simulink model "position_velocity_cascade"  (R2025b)
settings: configuration reference "MCConfiguration" (kept outside this file)
model workspace (MAT data in the model file):
  ControlOuter_Ts = Simulink.Parameter
  ControlOuter_Ts.Value = 0.001
  ControlOuter_Ts.Complexity = 'real'
  ControlOuter_Ts.Dimensions = [1 1]
  ControlOuter_Ts.DataType = 'auto'
  ControlOuter_Ts.DocUnits = 's'
undefined symbols (not defined in the file): ControlModes, DiscIntNeverNeededParam
libraries: simulink x12, slpidlib x3, simulink_extras x1
settings Model: DataDictionary=embeddedBoard_common.sldd  Creator=ascalzo  LastModifiedBy=rpumpo
settings ConfigSetRef: SourceName=MCConfiguration

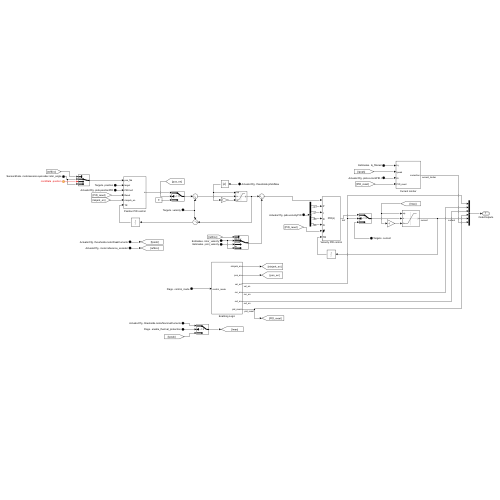
[thumbnail: Simulink's stored preview of the top-level diagram]
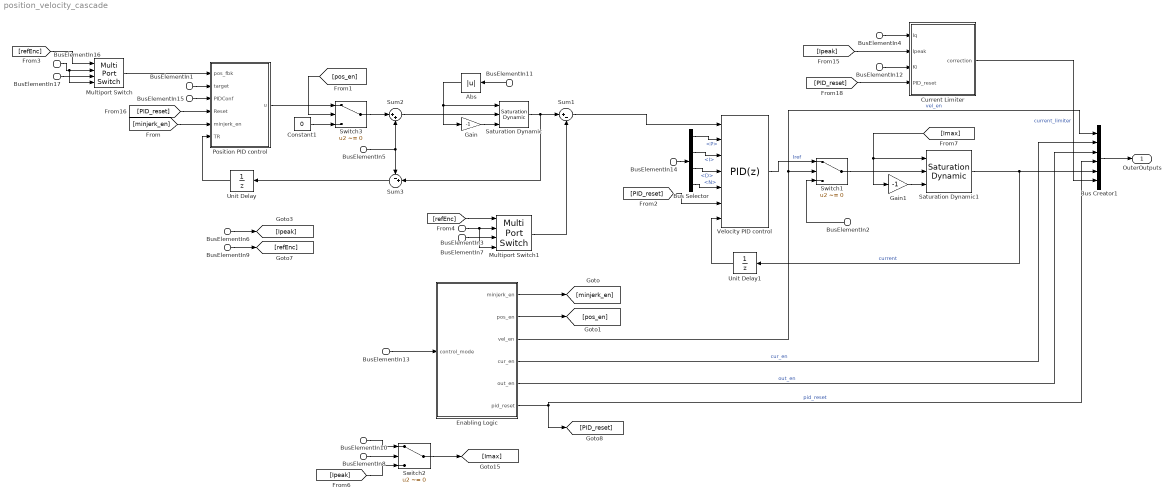
== system position_velocity_cascade ==
  BusElementIn3 : Inport  Description=velocity  PortName=Estimates  Element=rotor_velocity
  BusElementIn4 : Inport  Description=filtered motor current  PortName=Estimates  Element=Iq_filtered
  BusElementIn7 : Inport  Description=velocity  PortName=Estimates  Element=joint_velocity
  BusElementIn1 : Inport  Port=2  PortName=Targets  Element=position
  BusElementIn5 : Inport  Port=2  PortName=Targets  Element=velocity
  BusElementIn2 : Inport  Port=2  PortName=Targets  Element=current
  BusElementIn17 : Inport  Description=position encoder after gearbox  Port=3  PortName=JointData  Element=position
  BusElementIn11 : Inport  Description=Can be only non-negative  Port=4  PortName=ActuatorCfg  Element=thresholds.jntVelMax
  BusElementIn10 : Inport  Description=|  Port=4  PortName=ActuatorCfg  Element=thresholds.motorNominalCurrents
      | Current that can be kept for an indefinite period of time w/o damaging the motor
      | Expressed in [A] as all the internal computations are done this way
      | Can be only non-negative
  BusElementIn6 : Inport  Description=|  Port=4  PortName=ActuatorCfg  Element=thresholds.motorPeakCurrents
      | Current that can be applied for a short period of time
      | Expressed in [A] as all the internal computations are done this way
      | Can be only non-negative
  BusElementIn12 : Inport  Port=4  PortName=ActuatorCfg  Element=pids.currentPID.I
  BusElementIn14 : Inport  Port=4  PortName=ActuatorCfg  Element=pids.velocityPID
  BusElementIn15 : Inport  Port=4  PortName=ActuatorCfg  Element=pids.positionPID
  BusElementIn9 : Inport  Port=4  PortName=ActuatorCfg  Element=motor.reference_encoder
  BusElementIn16 : Inport  Description=Mechanical Angle before gearbox  Port=5  PortName=SensorsData  Element=motorsensors.qencoder.rotor_angle
  BusElementIn8 : Inport  Port=6  PortName=Flags  Element=enable_thermal_protection
  BusElementIn13 : Inport  Description=control mode  Port=6  PortName=Flags  Element=control_mode
  Abs : Abs  SaturateOnIntegerOverflow=off
  Bus Creator1 : BusCreator  Inputs=6  OutDataTypeStr=Bus: ControlOuterOutputs  NonVirtualBus=on
      settings: InheritFromInputs=off
  Bus Selector : BusSelector  OutputSignals=P,I,D,N
  Constant1 : Constant  Value=0  OutDataTypeStr=single  SampleTime=-1
  Current Limiter : Subsystem
  Enabling Logic : Subsystem
      settings: PortSchema="{\"entries\":[{\"content\":{\"sides\":[{\"content\":{},\"type\":\"ConnectorPlacement.EquallySpacedRectSide\",\"uuid\":\"90c86a81-f753-4d73-9375-c811c35622e9\"},{\"content\":{\"side\":\"RIGHT\"},\"type\":\"ConnectorPlacement.EquallySpacedRectSide\",\"uuid\":\"e17254f2-3c2d-4692-9f9e-d71cfac23eea\"},{\"content\":{\"connectorIds\":[\"Out1\",\"Out2\",\"Out3\",\"Out4\",\"Out5\",\"Out6\"],\"side\":\"TOP\"},\"type\":\"ConnectorPlacement.EquallySpacedRectSide\",\"uuid\":\"448c88e2-24ce-4de3-becf-cb98b7ef78f6\"},{\"content\":{\"connectorIds\":[\"In1\"],\"side\":\"BOTTOM\"},\"type\":\"ConnectorPlacement.EquallySpacedRectSide\",\"uuid\":\"8605ddaa-364c-411c-83c1-7277cb4d54d2\"}]},\"type\":\"ConnectorPlacement.EquallySpacedConnector\",\"uuid\":\"c1415ecc-9e2a-4576-ac3b-1f6784fd4a23\"}],\"packageUris\":[\"http://schema.mathworks.com/mf0/Connector/R2020b\"],\"version\":\"1.0\"}"
  Gain : Gain  Gain=-1
  Gain1 : Gain  Gain=-1
  Multiport Switch : MultiPortSwitch  DataPortOrder=Specify indices  Inputs=2  DataPortIndices={ ReferenceEncoder.Motor, ReferenceEncoder.Joint}  DataPortForDefault=Additional data port  SaturateOnIntegerOverflow=off  InputSameDT=off
  Multiport Switch1 : MultiPortSwitch  DataPortOrder=Specify indices  Inputs=2  DataPortIndices={ ReferenceEncoder.Motor, ReferenceEncoder.Joint}  DataPortForDefault=Additional data port  SaturateOnIntegerOverflow=off  InputSameDT=off
  Position PID control : Subsystem
  Saturation Dynamic : simulink/Discontinuities/Saturation Dynamic  OutMin=[]  OutMax=[]  OutDataTypeStr=Inherit: Same as second input  OutDataType=fixdt(1, 16)  OutScaling=2^-10  DoSatur=off
  Saturation Dynamic1 : simulink/Discontinuities/Saturation Dynamic  OutMin=[]  OutMax=[]  OutDataTypeStr=Inherit: Same as second input  OutDataType=fixdt(1, 16)  OutScaling=2^-10  DoSatur=off
  Sum1 : Sum  Inputs=|+-
  Sum2 : Sum  Inputs=|++
  Sum3 : Sum  Inputs=-+|
  Switch1 : Switch  Criteria=u2 ~= 0  SaturateOnIntegerOverflow=off  InputSameDT=off
  Switch2 : Switch  Criteria=u2 ~= 0  SaturateOnIntegerOverflow=off  InputSameDT=off
  Switch3 : Switch  Criteria=u2 ~= 0  SaturateOnIntegerOverflow=off  InputSameDT=off
  Unit Delay : UnitDelay  SampleTime=-1  HasFrameUpgradeWarning=on
  Unit Delay1 : UnitDelay  SampleTime=-1  HasFrameUpgradeWarning=on
  Velocity PID control : slpidlib/PID Controller  Controller=PID  Form=Parallel  TimeDomain=Discrete-time  UseExternalTs=off  SampleTime=-1  IntegratorMethod=Trapezoidal  FilterMethod=Trapezoidal  ControllerParametersSource=external  P=100  I=0  UseKiTs=off  D=0  UseExternalDerivativeSource=off  N=100  UseFilter=on  TunerSelectOption=Frequency Response Based  InitialConditionSource=internal  InitialConditionForIntegrator=0  InitialConditionForFilter=0  DifferentiatorICPrevScaledInput=0  ExternalReset=rising  TrackingMode=on  Kt=1  LimitOutput=off  SatLimitsSource=internal  UpperSaturationLimit=100  LowerSaturationLimit=-100  LinearizeAsGain=on  AntiWindupMode=clamping  Kb=1  LimitIntegrator=off  UpperIntegratorSaturationLimit=inf  LowerIntegratorSaturationLimit=-inf  POutMin=[]  POutMax=[]  IOutMin=[]  IOutMax=[]  DOutMin=[]  DOutMax=[]  NOutMin=[]  NOutMax=[]  SumOutMin=[]  SumOutMax=[]  SaturationOutMin=[]  SaturationOutMax=[]  PParamMin=[]  PParamMax=[]  IParamMin=[]  IParamMax=[]  DParamMin=[]  DParamMax=[]  NParamMin=[]  NParamMax=[]  KbParamMin=[]  KbParamMax=[]  KtParamMin=[]  KtParamMax=[]  KbOutMin=[]  KbOutMax=[]  KtOutMin=[]  KtOutMax=[]  IntegratorOutMin=[]  IntegratorOutMax=[]  FilterOutMin=[]  FilterOutMax=[]  SumI1OutMin=[]  SumI1OutMax=[]  SumI2OutMin=[]  SumI2OutMax=[]  SumI3OutMin=[]  SumI3OutMax=[]  SumI4OutMin=[]  SumI4OutMax=[]  SumDOutMin=[]  SumDOutMax=[]  DifferentiatorOutMin=[]  DifferentiatorOutMax=[]  FilterDiffOutCoefMin=[]  FilterDiffOutCoefMax=[]  ReciprocalOutMin=[]  ReciprocalOutMax=[]  SumDenOutMin=[]  SumDenOutMax=[]  SumNumOutMin=[]  SumNumOutMax=[]  DivideOutMin=[]  DivideOutMax=[]  UdiffTsProdOutMin=[]  UdiffTsProdOutMax=[]  NTsProdOutMin=[]  NTsProdOutMax=[]  UintegralTsProdOutMin=[]  UintegralTsProdOutMax=[]  UngainTsProdOutMin=[]  UngainTsProdOutMax=[]  ClampingZeroOutDataTypeStr=Inherit: Inherit via back propagation  ClampingZeroOutMin=[]  ClampingZeroOutMax=[]  FilterDenConstantOutDataTypeStr=Inherit: Inherit via back propagation  FilterDenConstantOutMin=[]  FilterDenConstantOutMax=[]  PCopyOutDataTypeStr=Inherit: Inherit via back propagation  PCopyOutMin=[]  PCopyOutMax=[]  NCopyOutDataTypeStr=Inherit: Inherit via back propagation  NCopyOutMin=[]  NCopyOutMax=[]  IntegratorContinuousStateAttributes=''  IntegratorStateMustResolveToSignalObject=off  IntegratorRTWStateStorageClass=Auto  FilterContinuousStateAttributes=''  FilterStateMustResolveToSignalObject=off  FilterRTWStateStorageClass=Auto  ParallelPVariant=ExternalParameters  IdealPVariant=Disabled  IVariant=ExternalParameters  DVariant=ExternalParameters  IntegratorVariant=Discrete  SatVariant=Disabled  AWVariant=Passthrough  PCopyVariant=Disabled  TRVariant=Enabled  FdbkBlocksVariant=Feedback  IdealPFdbkVariant=Passthrough  SatFdbkVariant=Passthrough  DerivativeFilterVariant=TrapezoidalFilter  NVariant=ExternalParameters  NCopyVariant=ExternalParameters  FilterICVariant=InternalICsFilter  IntegratorICVariant=InternalICs  ExternalResetVariant=ExternalReset  TRSumVariant=TrackingMode  SumFdbkVariant=Enabled  SumVariant=Sum_PID  TsampFilterVariant=InternalTs  TsampNgainVariant=Passthrough  TsampIntegralVariant=Disabled_SignalSpec  ExternalSaturationOutDataTypeStr=Inherit: Same as second input  DerivativeSourceVariant=ErrorSignal  PreIntVariant=InternalPreInt
  OuterOutputs : Outport  OutDataTypeStr=Bus: ControlOuterOutputs  BusOutputAsStruct=on
  wires:
  [PID_reset] -> Velocity PID control/6
  BusElementIn14/1 -> Bus Selector/1
  Sum2/1 -> Saturation Dynamic/2
  Switch3/1 -> Sum2/1
  Constant1/1 -> Switch3/3
  BusElementIn15/1 -> Position PID control/3(PIDConf)
  BusElementIn1/1 -> Position PID control/2(target)
  [PID_reset] -> Position PID control/4(Reset)
  Position PID control/1(u) -> Switch3/1
  BusElementIn5/1 -> Sum3/1, Sum2/2
  Saturation Dynamic/1 -> Sum1/1, Sum3/2
  Sum3/1 -> Unit Delay/1
  Unit Delay/1 -> Position PID control/6(TR)
  Enabling Logic/1(minjerk_en) -> [minjerk_en]
  Enabling Logic/2(pos_en) -> [pos_en]
  [minjerk_en] -> Position PID control/5(minjerk_en)
  [pos_en] -> Switch3/2
  Enabling Logic/3(vel_en) -> Switch1/2, Bus Creator1/1  "vel_en"
  Enabling Logic/4(cur_en) -> Bus Creator1/2  "cur_en"
  Enabling Logic/5(out_en) -> Bus Creator1/3  "out_en"
  Bus Creator1/1 -> OuterOutputs/1
  BusElementIn13/1 -> Enabling Logic/1(control_mode)
  BusElementIn11/1 -> Abs/1
  Abs/1 -> Gain/1, Saturation Dynamic/1
  Gain/1 -> Saturation Dynamic/3
  Unit Delay1/1 -> Velocity PID control/7
  Velocity PID control/1 -> Switch1/1  "Iref"
  Switch1/1 -> Saturation Dynamic1/2
  BusElementIn2/1 -> Switch1/3
  Gain1/1 -> Saturation Dynamic1/3
  [Imax] -> Saturation Dynamic1/1, Gain1/1
  BusElementIn4/1 -> Current Limiter/1(Iq)
  [Ipeak] -> Current Limiter/2(Ipeak)
  [PID_reset] -> Current Limiter/4(PID_reset)
  BusElementIn12/1 -> Current Limiter/3(Ki)
  Sum1/1 -> Velocity PID control/1
  Enabling Logic/6(pid_reset) -> Bus Creator1/4, [PID_reset]  "pid_reset"
  Saturation Dynamic1/1 -> Bus Creator1/5, Unit Delay1/1  "current"
  Current Limiter/1(correction) -> Bus Creator1/6  "current_limiter"
  [Ipeak] -> Switch2/3
  BusElementIn10/1 -> Switch2/1
  BusElementIn8/1 -> Switch2/2
  Switch2/1 -> [Imax]
  Multiport Switch/1 -> Position PID control/1(pos_fbk)
  [refEnc] -> Multiport Switch/1
  BusElementIn17/1 -> Multiport Switch/3
  BusElementIn16/1 -> Multiport Switch/4, Multiport Switch/2
  BusElementIn3/1 -> Multiport Switch1/4, Multiport Switch1/2
  BusElementIn7/1 -> Multiport Switch1/3
  Multiport Switch1/1 -> Sum1/2
  [refEnc] -> Multiport Switch1/1
  BusElementIn9/1 -> [refEnc]
  BusElementIn6/1 -> [Ipeak]
  Bus Selector/1 -> Velocity PID control/2  "<P>"
  Bus Selector/2 -> Velocity PID control/3  "<I>"
  Bus Selector/3 -> Velocity PID control/4  "<D>"
  Bus Selector/4 -> Velocity PID control/5  "<N>"

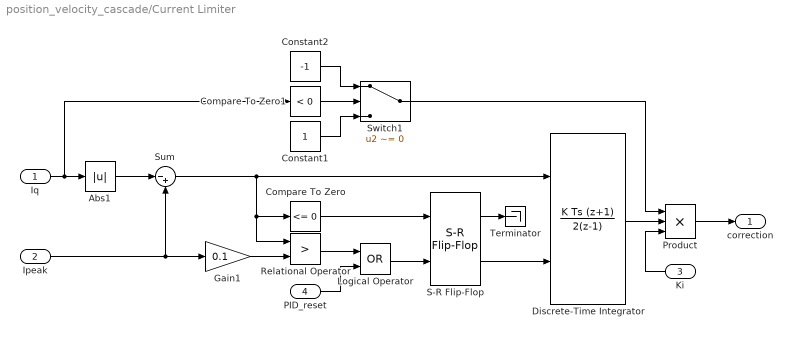
== system position_velocity_cascade/Current Limiter ==
  Iq : Inport
  Ipeak : Inport  Port=2
  Ki : Inport  Port=3
  PID_reset : Inport  Port=4
  Abs1 : Abs  SaturateOnIntegerOverflow=off
  Compare To Zero : simulink/Logic and Bit Operations/Compare To Zero  relop=<=  OutDataTypeStr=boolean
  Compare To Zero1 : simulink/Logic and Bit Operations/Compare To Zero  relop=<  OutDataTypeStr=boolean
  Constant1 : Constant  OutDataTypeStr=single
  Constant2 : Constant  Value=-1  OutDataTypeStr=single
  Discrete-Time Integrator : DiscreteIntegrator  IntegratorMethod=Integration: Trapezoidal  ExternalReset=level  SampleTime=-1  ICPrevOutput=DiscIntNeverNeededParam  ICPrevScaledInput=DiscIntNeverNeededParam
  Gain1 : Gain  Gain=0.1  OutDataTypeStr=single
  Logical Operator : Logic  Operator=OR  AllPortsSameDT=off  OutDataTypeStr=boolean
  Product : Product  Inputs=3
  Relational Operator : RelationalOperator  Operator=>  OutDataTypeStr=boolean  RndMeth=Simplest  InputSameDT=off
  S-R Flip-Flop : simulink_extras/Flip Flops/S-R Flip-Flop  initial_condition=0
  Sum : Sum  Inputs=|-+
  Switch1 : Switch  Criteria=u2 ~= 0  SaturateOnIntegerOverflow=off  InputSameDT=off
  Terminator : Terminator
  correction : Outport
  wires:
  Sum/1 -> Relational Operator/1, Compare To Zero/1, Discrete-Time Integrator/1
  Iq/1 -> Compare To Zero1/1, Abs1/1
  Product/1 -> correction/1
  Compare To Zero/1 -> S-R Flip-Flop/1
  Abs1/1 -> Sum/1
  Ipeak/1 -> Gain1/1, Sum/2
  Gain1/1 -> Relational Operator/2
  S-R Flip-Flop/2 -> Discrete-Time Integrator/2
  S-R Flip-Flop/1 -> Terminator/1
  Relational Operator/1 -> Logical Operator/1
  Logical Operator/1 -> S-R Flip-Flop/2
  PID_reset/1 -> Logical Operator/2
  Discrete-Time Integrator/1 -> Product/2
  Ki/1 -> Product/3
  Compare To Zero1/1 -> Switch1/2
  Constant2/1 -> Switch1/1
  Constant1/1 -> Switch1/3
  Switch1/1 -> Product/1

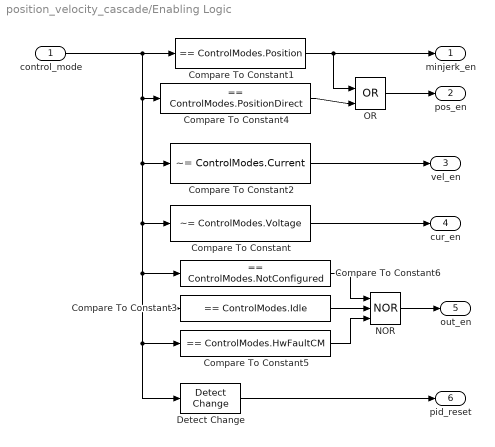
== system position_velocity_cascade/Enabling Logic ==
  control_mode : Inport
  Compare To Constant : simulink/Logic and Bit Operations/Compare To Constant  relop=~=  const=ControlModes.Voltage  OutDataTypeStr=boolean
  Compare To Constant1 : simulink/Logic and Bit Operations/Compare To Constant  relop===  const=ControlModes.Position  OutDataTypeStr=boolean
  Compare To Constant2 : simulink/Logic and Bit Operations/Compare To Constant  relop=~=  const=ControlModes.Current  OutDataTypeStr=boolean
  Compare To Constant3 : simulink/Logic and Bit Operations/Compare To Constant  relop===  const=ControlModes.Idle  OutDataTypeStr=boolean
  Compare To Constant4 : simulink/Logic and Bit Operations/Compare To Constant  relop===  const=ControlModes.PositionDirect  OutDataTypeStr=boolean
  Compare To Constant5 : simulink/Logic and Bit Operations/Compare To Constant  relop===  const=ControlModes.HwFaultCM  OutDataTypeStr=boolean
  Compare To Constant6 : simulink/Logic and Bit Operations/Compare To Constant  relop===  const=ControlModes.NotConfigured  OutDataTypeStr=boolean
  Detect Change : simulink/Logic and Bit Operations/Detect Change  vinit=ControlModes.Idle  OutDataTypeStr=boolean
  NOR : Logic  Operator=NOR  Inputs=3  IconShape=distinctive  AllPortsSameDT=off  OutDataTypeStr=boolean
  OR : Logic  Operator=OR  IconShape=distinctive  AllPortsSameDT=off  OutDataTypeStr=boolean
  minjerk_en : Outport
  pos_en : Outport  Port=2
  vel_en : Outport  Port=3
  cur_en : Outport  Port=4
  out_en : Outport  Port=5
  pid_reset : Outport  Port=6
  wires:
  Compare To Constant4/1 -> OR/2
  control_mode/1 -> Detect Change/1, Compare To Constant5/1, Compare To Constant3/1, Compare To Constant6/1, Compare To Constant/1, Compare To Constant2/1, Compare To Constant4/1, Compare To Constant1/1
  Compare To Constant1/1 -> OR/1, minjerk_en/1
  OR/1 -> pos_en/1
  Compare To Constant5/1 -> NOR/3
  Compare To Constant6/1 -> NOR/1
  Compare To Constant3/1 -> NOR/2
  Detect Change/1 -> pid_reset/1
  Compare To Constant2/1 -> vel_en/1
  Compare To Constant/1 -> cur_en/1
  NOR/1 -> out_en/1

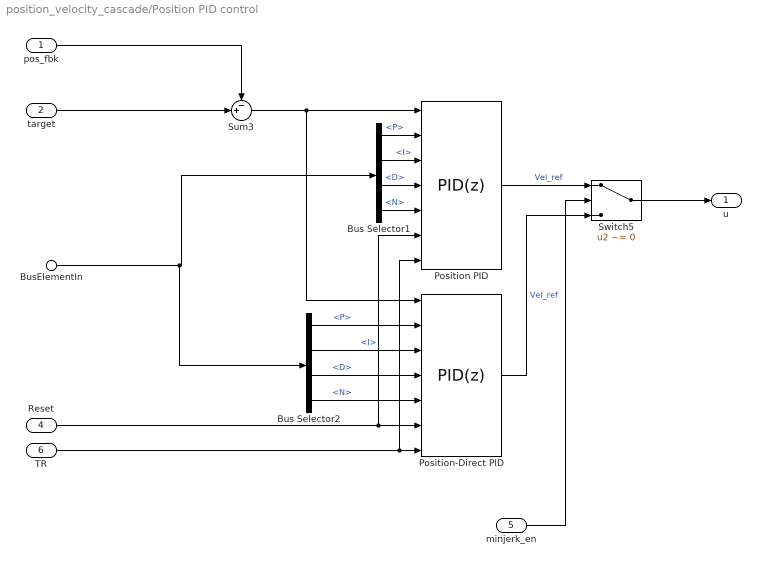
== system position_velocity_cascade/Position PID control ==
  pos_fbk : Inport
  target : Inport  Port=2
  BusElementIn : Inport  Port=3  PortName=PIDConf
  Reset : Inport  Port=4
  minjerk_en : Inport  Port=5
  TR : Inport  Port=6
  Bus Selector1 : BusSelector  OutputSignals=P,I,D,N
  Bus Selector2 : BusSelector  OutputSignals=P,I,D,N
  Position PID : slpidlib/PID Controller  Controller=PID  Form=Parallel  TimeDomain=Discrete-time  UseExternalTs=off  SampleTime=-1  IntegratorMethod=Trapezoidal  FilterMethod=Trapezoidal  ControllerParametersSource=external  P=1  I=1  UseKiTs=off  D=0  UseExternalDerivativeSource=off  N=100  UseFilter=on  TunerSelectOption=Frequency Response Based  InitialConditionSource=internal  InitialConditionForIntegrator=0  InitialConditionForFilter=0  DifferentiatorICPrevScaledInput=0  ExternalReset=rising  TrackingMode=on  Kt=1  LimitOutput=off  SatLimitsSource=internal  UpperSaturationLimit=100  LowerSaturationLimit=-100  LinearizeAsGain=on  AntiWindupMode=clamping  Kb=1  LimitIntegrator=off  UpperIntegratorSaturationLimit=inf  LowerIntegratorSaturationLimit=-inf  POutMin=[]  POutMax=[]  IOutMin=[]  IOutMax=[]  DOutMin=[]  DOutMax=[]  NOutMin=[]  NOutMax=[]  SumOutMin=[]  SumOutMax=[]  SaturationOutMin=[]  SaturationOutMax=[]  PParamMin=[]  PParamMax=[]  IParamMin=[]  IParamMax=[]  DParamMin=[]  DParamMax=[]  NParamMin=[]  NParamMax=[]  KbParamMin=[]  KbParamMax=[]  KtParamMin=[]  KtParamMax=[]  KbOutMin=[]  KbOutMax=[]  KtOutMin=[]  KtOutMax=[]  IntegratorOutMin=[]  IntegratorOutMax=[]  FilterOutMin=[]  FilterOutMax=[]  SumI1OutMin=[]  SumI1OutMax=[]  SumI2OutMin=[]  SumI2OutMax=[]  SumI3OutMin=[]  SumI3OutMax=[]  SumI4OutMin=[]  SumI4OutMax=[]  SumDOutMin=[]  SumDOutMax=[]  DifferentiatorOutMin=[]  DifferentiatorOutMax=[]  FilterDiffOutCoefMin=[]  FilterDiffOutCoefMax=[]  ReciprocalOutMin=[]  ReciprocalOutMax=[]  SumDenOutMin=[]  SumDenOutMax=[]  SumNumOutMin=[]  SumNumOutMax=[]  DivideOutMin=[]  DivideOutMax=[]  UdiffTsProdOutMin=[]  UdiffTsProdOutMax=[]  NTsProdOutMin=[]  NTsProdOutMax=[]  UintegralTsProdOutMin=[]  UintegralTsProdOutMax=[]  UngainTsProdOutMin=[]  UngainTsProdOutMax=[]  ClampingZeroOutDataTypeStr=Inherit: Inherit via back propagation  ClampingZeroOutMin=[]  ClampingZeroOutMax=[]  FilterDenConstantOutDataTypeStr=Inherit: Inherit via back propagation  FilterDenConstantOutMin=[]  FilterDenConstantOutMax=[]  PCopyOutDataTypeStr=Inherit: Inherit via back propagation  PCopyOutMin=[]  PCopyOutMax=[]  NCopyOutDataTypeStr=Inherit: Inherit via back propagation  NCopyOutMin=[]  NCopyOutMax=[]  IntegratorContinuousStateAttributes=''  IntegratorStateMustResolveToSignalObject=off  IntegratorRTWStateStorageClass=Auto  FilterContinuousStateAttributes=''  FilterStateMustResolveToSignalObject=off  FilterRTWStateStorageClass=Auto  ParallelPVariant=ExternalParameters  IdealPVariant=Disabled  IVariant=ExternalParameters  DVariant=ExternalParameters  IntegratorVariant=Discrete  SatVariant=Disabled  AWVariant=Passthrough  PCopyVariant=Disabled  TRVariant=Enabled  FdbkBlocksVariant=Feedback  IdealPFdbkVariant=Passthrough  SatFdbkVariant=Passthrough  DerivativeFilterVariant=TrapezoidalFilter  NVariant=ExternalParameters  NCopyVariant=ExternalParameters  FilterICVariant=InternalICsFilter  IntegratorICVariant=InternalICs  ExternalResetVariant=ExternalReset  TRSumVariant=TrackingMode  SumFdbkVariant=Enabled  SumVariant=Sum_PID  TsampFilterVariant=InternalTs  TsampNgainVariant=Passthrough  TsampIntegralVariant=Disabled_SignalSpec  ExternalSaturationOutDataTypeStr=Inherit: Same as second input  DerivativeSourceVariant=ErrorSignal  PreIntVariant=InternalPreInt
  Position-Direct PID : slpidlib/PID Controller  Controller=PID  Form=Parallel  TimeDomain=Discrete-time  UseExternalTs=off  SampleTime=-1  IntegratorMethod=Trapezoidal  FilterMethod=Trapezoidal  ControllerParametersSource=external  P=1  I=1  UseKiTs=off  D=0  UseExternalDerivativeSource=off  N=100  UseFilter=on  TunerSelectOption=Frequency Response Based  InitialConditionSource=internal  InitialConditionForIntegrator=0  InitialConditionForFilter=0  DifferentiatorICPrevScaledInput=0  ExternalReset=rising  TrackingMode=on  Kt=1  LimitOutput=off  SatLimitsSource=internal  UpperSaturationLimit=100  LowerSaturationLimit=-100  LinearizeAsGain=on  AntiWindupMode=clamping  Kb=1  LimitIntegrator=off  UpperIntegratorSaturationLimit=inf  LowerIntegratorSaturationLimit=-inf  POutMin=[]  POutMax=[]  IOutMin=[]  IOutMax=[]  DOutMin=[]  DOutMax=[]  NOutMin=[]  NOutMax=[]  SumOutMin=[]  SumOutMax=[]  SaturationOutMin=[]  SaturationOutMax=[]  PParamMin=[]  PParamMax=[]  IParamMin=[]  IParamMax=[]  DParamMin=[]  DParamMax=[]  NParamMin=[]  NParamMax=[]  KbParamMin=[]  KbParamMax=[]  KtParamMin=[]  KtParamMax=[]  KbOutMin=[]  KbOutMax=[]  KtOutMin=[]  KtOutMax=[]  IntegratorOutMin=[]  IntegratorOutMax=[]  FilterOutMin=[]  FilterOutMax=[]  SumI1OutMin=[]  SumI1OutMax=[]  SumI2OutMin=[]  SumI2OutMax=[]  SumI3OutMin=[]  SumI3OutMax=[]  SumI4OutMin=[]  SumI4OutMax=[]  SumDOutMin=[]  SumDOutMax=[]  DifferentiatorOutMin=[]  DifferentiatorOutMax=[]  FilterDiffOutCoefMin=[]  FilterDiffOutCoefMax=[]  ReciprocalOutMin=[]  ReciprocalOutMax=[]  SumDenOutMin=[]  SumDenOutMax=[]  SumNumOutMin=[]  SumNumOutMax=[]  DivideOutMin=[]  DivideOutMax=[]  UdiffTsProdOutMin=[]  UdiffTsProdOutMax=[]  NTsProdOutMin=[]  NTsProdOutMax=[]  UintegralTsProdOutMin=[]  UintegralTsProdOutMax=[]  UngainTsProdOutMin=[]  UngainTsProdOutMax=[]  ClampingZeroOutDataTypeStr=Inherit: Inherit via back propagation  ClampingZeroOutMin=[]  ClampingZeroOutMax=[]  FilterDenConstantOutDataTypeStr=Inherit: Inherit via back propagation  FilterDenConstantOutMin=[]  FilterDenConstantOutMax=[]  PCopyOutDataTypeStr=Inherit: Inherit via back propagation  PCopyOutMin=[]  PCopyOutMax=[]  NCopyOutDataTypeStr=Inherit: Inherit via back propagation  NCopyOutMin=[]  NCopyOutMax=[]  IntegratorContinuousStateAttributes=''  IntegratorStateMustResolveToSignalObject=off  IntegratorRTWStateStorageClass=Auto  FilterContinuousStateAttributes=''  FilterStateMustResolveToSignalObject=off  FilterRTWStateStorageClass=Auto  ParallelPVariant=ExternalParameters  IdealPVariant=Disabled  IVariant=ExternalParameters  DVariant=ExternalParameters  IntegratorVariant=Discrete  SatVariant=Disabled  AWVariant=Passthrough  PCopyVariant=Disabled  TRVariant=Enabled  FdbkBlocksVariant=Feedback  IdealPFdbkVariant=Passthrough  SatFdbkVariant=Passthrough  DerivativeFilterVariant=TrapezoidalFilter  NVariant=ExternalParameters  NCopyVariant=ExternalParameters  FilterICVariant=InternalICsFilter  IntegratorICVariant=InternalICs  ExternalResetVariant=ExternalReset  TRSumVariant=TrackingMode  SumFdbkVariant=Enabled  SumVariant=Sum_PID  TsampFilterVariant=InternalTs  TsampNgainVariant=Passthrough  TsampIntegralVariant=Disabled_SignalSpec  ExternalSaturationOutDataTypeStr=Inherit: Same as second input  DerivativeSourceVariant=ErrorSignal  PreIntVariant=InternalPreInt
  Sum3 : Sum  Inputs=-+|
  Switch5 : Switch  Criteria=u2 ~= 0  SaturateOnIntegerOverflow=off  InputSameDT=off
  u : Outport
  wires:
  Bus Selector2/3 -> Position-Direct PID/4  "<D>"
  Bus Selector2/1 -> Position-Direct PID/2  "<P>"
  Switch5/1 -> u/1
  Sum3/1 -> Position-Direct PID/1, Position PID/1
  Bus Selector2/4 -> Position-Direct PID/5  "<N>"
  target/1 -> Sum3/2
  pos_fbk/1 -> Sum3/1
  Bus Selector1/3 -> Position PID/4  "<D>"
  Position PID/1 -> Switch5/1  "Vel_ref"
  Bus Selector1/2 -> Position PID/3  "<I>"
  Bus Selector1/4 -> Position PID/5  "<N>"
  Bus Selector2/2 -> Position-Direct PID/3  "<I>"
  Bus Selector1/1 -> Position PID/2  "<P>"
  Reset/1 -> Position PID/6, Position-Direct PID/6
  Position-Direct PID/1 -> Switch5/3  "Vel_ref"
  minjerk_en/1 -> Switch5/2
  TR/1 -> Position PID/7, Position-Direct PID/7
  BusElementIn/1 -> Bus Selector2/1, Bus Selector1/1
